simulink model "H03_ERR"  (R2026a)
settings: Solver=VariableStepAuto  MaxStep=tau/25
InitFcn:
  | K = 5;
  | tau = 0.125;
settings Model: Creator=Szalay  LastModifiedBy=Szalay

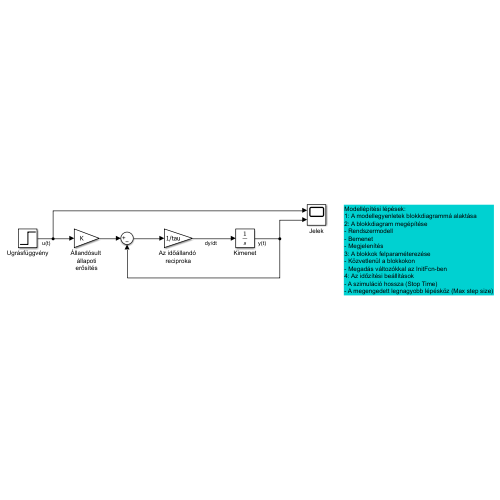
[thumbnail: Simulink's stored preview of the top-level diagram]
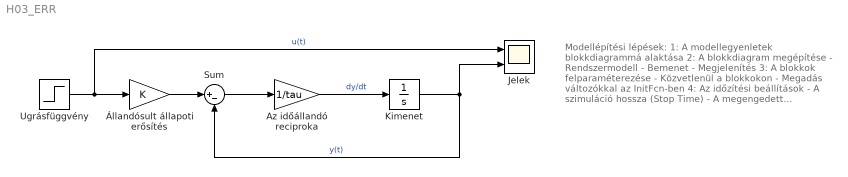
== system H03_ERR ==
  note: Modellépítési lépések:
      | 1: A modellegyenletek blokkdiagrammá alaktása
      | 2: A blokkdiagram megépítése
      | - Rendszermodell
      | - Bemenet
      | - Megjelenítés
      | 3: A blokkok felparaméterezése
      | - Közvetlenül a blokkokon
      | - Megadás változókkal az InitFcn-ben
      | 4: Az időzítési beállítások
      | - A szimuláció hossza (Stop Time)
      | - A megengedett legnagyobb lépésköz (Max step size)
  Az időállandó reciproka : Gain  Gain=1/tau
  Jelek : Scope  NumInputPorts=2
      settings: ActiveDisplayYMinimum=-0.6249999987117788  ActiveDisplayYMaximum=5.62499998840601
  Kimenet : Integrator  InitialCondition=0.5
  Sum : Sum  Inputs=|+-
  Ugrásfüggvény : Step  Time=5  SampleTime=0
  Állandósult állapoti erősítés : Gain  Gain=K
  wires:
  Kimenet/1 -> Sum/2, Jelek/2  "y(t)"
  Az időállandó reciproka/1 -> Kimenet/1  "dy/dt"
  Sum/1 -> Az időállandó reciproka/1
  Állandósult állapoti erősítés/1 -> Sum/1
  Ugrásfüggvény/1 -> Jelek/1, Állandósult állapoti erősítés/1  "u(t)"
